simulink model "ControlSystemSimulation"  (R2023a)
settings: Solver=FixedStepDiscrete  StartTime=0.0  StopTime=60  FixedStep=Ts  RelTol=1e-3
undefined symbols (not defined in the file): A_eso, Aa, Ad, b0, B_eso, Ba, Bd, C_eso, Ca, Cd, D_eso, deltaAd, deltay, DiscIntNeverNeededParam, Ed, k_current, k_disturb, k_MN, k_of, Kc, L, N, nr, p_MN, p_of, T, Ts, vmax, wsin, z_MN, z_of
libraries: simulink x5, cstblocks x4, slpidlib x2
settings Model: Creator=jueqi  LastModifiedBy=13529

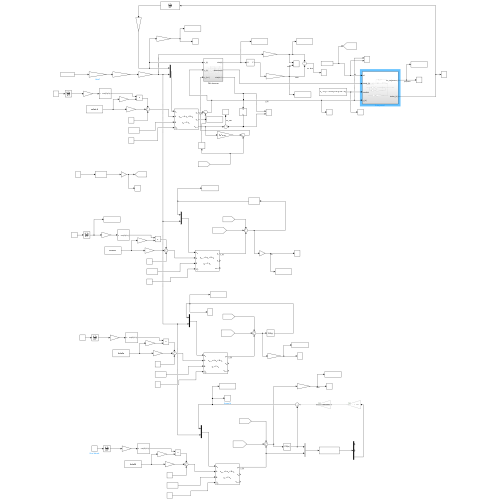
[thumbnail: Simulink's stored preview of the top-level diagram]
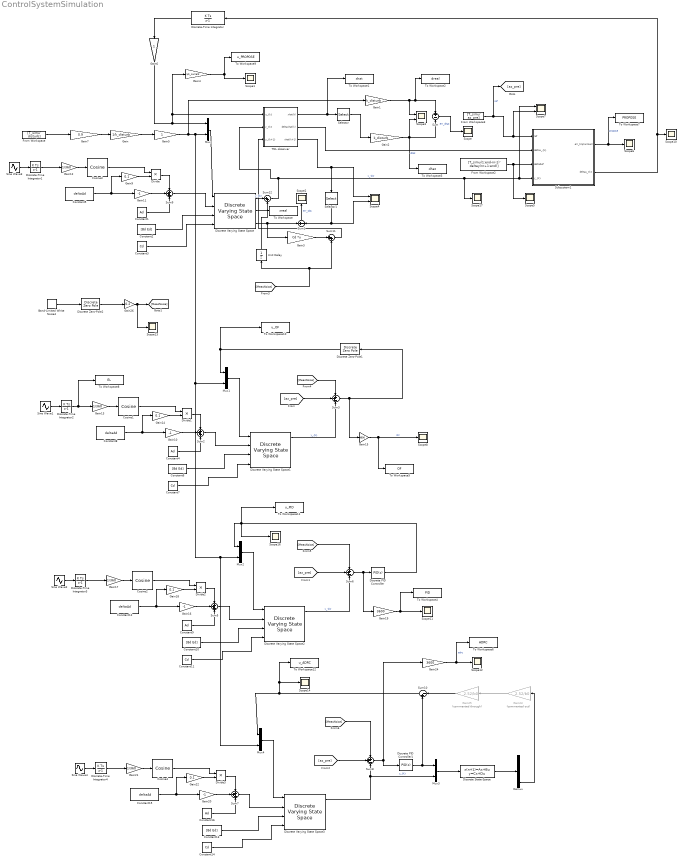
== system ControlSystemSimulation ==
  Band-Limited White Noise4 : simulink/Sources/Band-Limited White Noise  Cov=[1e-12]  Ts=Ts  seed=[23341]
  Constant{1,4,9,16} (4 alike) : Constant  Value=Ad
  Constant{2,6,10,13} (4 alike) : Constant  Value=[Bd Ed]
  Constant{3,7,11,14} (4 alike) : Constant  Value=Cd  VectorParams1D=off
  Constant{5,8,12,15} (4 alike) : Constant  Value=deltaAd
  Cosine{1..4} (4 alike) : simulink/Lookup Tables/Cosine  Formula=cos(2*pi*u)  NumDataPoints=(2^5)+1  OutputWordLength=16  InternalRulePriority=Speed
  Demux : Demux  Outputs=3
  Discrete Zero-Pole1 : DiscreteZeroPole  Zeros=z_of  Poles=p_of  Gain=k_of  SampleTime=Ts
  Discrete Zero-Pole2 : DiscreteZeroPole  Zeros=z_MN  Poles=p_MN  Gain=k_MN  SampleTime=Ts
  Discrete PID Controller : slpidlib/PID Controller  Controller=PID  Form=Parallel  TimeDomain=Discrete-time  UseExternalTs=off  SampleTime=-1  IntegratorMethod=Forward Euler  FilterMethod=Forward Euler  ControllerParametersSource=internal  P=25  I=0.3  UseKiTs=off  D=5  N=100  UseFilter=on  TunerSelectOption=Transfer Function Based (PID Tuner App)  InitialConditionSource=internal  InitialConditionForIntegrator=0  InitialConditionForFilter=0  DifferentiatorICPrevScaledInput=0  ExternalReset=none  TrackingMode=off  Kt=1  LimitOutput=off  SatLimitsSource=internal  UpperSaturationLimit=inf  LowerSaturationLimit=-inf  LinearizeAsGain=off  AntiWindupMode=none  Kb=1  LimitIntegrator=off  UpperIntegratorSaturationLimit=inf  LowerIntegratorSaturationLimit=-inf  POutMin=[]  POutMax=[]  IOutMin=[]  IOutMax=[]  DOutMin=[]  DOutMax=[]  NOutMin=[]  NOutMax=[]  SumOutMin=[]  SumOutMax=[]  SaturationOutMin=[]  SaturationOutMax=[]  PParamMin=[]  PParamMax=[]  IParamMin=[]  IParamMax=[]  DParamMin=[]  DParamMax=[]  NParamMin=[]  NParamMax=[]  KbParamMin=[]  KbParamMax=[]  KtParamMin=[]  KtParamMax=[]  KbOutMin=[]  KbOutMax=[]  KtOutMin=[]  KtOutMax=[]  IntegratorOutMin=[]  IntegratorOutMax=[]  FilterOutMin=[]  FilterOutMax=[]  SumI1OutMin=[]  SumI1OutMax=[]  SumI2OutMin=[]  SumI2OutMax=[]  SumI3OutMin=[]  SumI3OutMax=[]  SumI4OutMin=[]  SumI4OutMax=[]  SumDOutMin=[]  SumDOutMax=[]  DifferentiatorOutMin=[]  DifferentiatorOutMax=[]  FilterDiffOutCoefMin=[]  FilterDiffOutCoefMax=[]  ReciprocalOutMin=[]  ReciprocalOutMax=[]  SumDenOutMin=[]  SumDenOutMax=[]  SumNumOutMin=[]  SumNumOutMax=[]  DivideOutMin=[]  DivideOutMax=[]  UdiffTsProdOutMin=[]  UdiffTsProdOutMax=[]  NTsProdOutMin=[]  NTsProdOutMax=[]  UintegralTsProdOutMin=[]  UintegralTsProdOutMax=[]  UngainTsProdOutMin=[]  UngainTsProdOutMax=[]  ClampingZeroOutDataTypeStr=Inherit: Inherit via back propagation  ClampingZeroOutMin=[]  ClampingZeroOutMax=[]  FilterDenConstantOutDataTypeStr=Inherit: Inherit via back propagation  FilterDenConstantOutMin=[]  FilterDenConstantOutMax=[]  PCopyOutDataTypeStr=Inherit: Inherit via back propagation  PCopyOutMin=[]  PCopyOutMax=[]  NCopyOutDataTypeStr=Inherit: Inherit via back propagation  NCopyOutMin=[]  NCopyOutMax=[]  IntegratorContinuousStateAttributes=''  IntegratorStateMustResolveToSignalObject=off  IntegratorRTWStateStorageClass=Auto  FilterContinuousStateAttributes=''  FilterStateMustResolveToSignalObject=off  FilterRTWStateStorageClass=Auto  ParallelPVariant=InternalParameters  IdealPVariant=Disabled  IVariant=InternalParameters  DVariant=InternalParameters  IntegratorVariant=Discrete  SatVariant=Disabled  AWVariant=Passthrough  PCopyVariant=Disabled  TRVariant=Disabled  FdbkBlocksVariant=Forward  IdealPFdbkVariant=Disabled  SatFdbkVariant=Disabled  DerivativeFilterVariant=ForwardEulerFilter  NVariant=InternalParameters  NCopyVariant=Disabled  FilterICVariant=InternalICsFilter  IntegratorICVariant=InternalICs  ExternalResetVariant=Disabled  TRSumVariant=Passthrough  SumFdbkVariant=Disabled  SumVariant=Sum_PID  TsampFilterVariant=InternalTs  TsampNgainVariant=Passthrough  TsampIntegralVariant=Disabled_SignalSpec  ExternalSaturationOutDataTypeStr=Inherit: Same as second input
      settings: LibrarySourceBlock=simulink/Discrete/Discrete PID Controller
  Discrete PID Controller1 : slpidlib/PID Controller  Controller=PID  Form=Parallel  TimeDomain=Discrete-time  UseExternalTs=off  SampleTime=-1  IntegratorMethod=Forward Euler  FilterMethod=Forward Euler  ControllerParametersSource=internal  P=150  I=1  UseKiTs=off  D=15  N=100  UseFilter=on  TunerSelectOption=Transfer Function Based (PID Tuner App)  InitialConditionSource=internal  InitialConditionForIntegrator=0  InitialConditionForFilter=0  DifferentiatorICPrevScaledInput=0  ExternalReset=none  TrackingMode=off  Kt=1  LimitOutput=off  SatLimitsSource=internal  UpperSaturationLimit=inf  LowerSaturationLimit=-inf  LinearizeAsGain=off  AntiWindupMode=none  Kb=1  LimitIntegrator=off  UpperIntegratorSaturationLimit=inf  LowerIntegratorSaturationLimit=-inf  POutMin=[]  POutMax=[]  IOutMin=[]  IOutMax=[]  DOutMin=[]  DOutMax=[]  NOutMin=[]  NOutMax=[]  SumOutMin=[]  SumOutMax=[]  SaturationOutMin=[]  SaturationOutMax=[]  PParamMin=[]  PParamMax=[]  IParamMin=[]  IParamMax=[]  DParamMin=[]  DParamMax=[]  NParamMin=[]  NParamMax=[]  KbParamMin=[]  KbParamMax=[]  KtParamMin=[]  KtParamMax=[]  KbOutMin=[]  KbOutMax=[]  KtOutMin=[]  KtOutMax=[]  IntegratorOutMin=[]  IntegratorOutMax=[]  FilterOutMin=[]  FilterOutMax=[]  SumI1OutMin=[]  SumI1OutMax=[]  SumI2OutMin=[]  SumI2OutMax=[]  SumI3OutMin=[]  SumI3OutMax=[]  SumI4OutMin=[]  SumI4OutMax=[]  SumDOutMin=[]  SumDOutMax=[]  DifferentiatorOutMin=[]  DifferentiatorOutMax=[]  FilterDiffOutCoefMin=[]  FilterDiffOutCoefMax=[]  ReciprocalOutMin=[]  ReciprocalOutMax=[]  SumDenOutMin=[]  SumDenOutMax=[]  SumNumOutMin=[]  SumNumOutMax=[]  DivideOutMin=[]  DivideOutMax=[]  UdiffTsProdOutMin=[]  UdiffTsProdOutMax=[]  NTsProdOutMin=[]  NTsProdOutMax=[]  UintegralTsProdOutMin=[]  UintegralTsProdOutMax=[]  UngainTsProdOutMin=[]  UngainTsProdOutMax=[]  ClampingZeroOutDataTypeStr=Inherit: Inherit via back propagation  ClampingZeroOutMin=[]  ClampingZeroOutMax=[]  FilterDenConstantOutDataTypeStr=Inherit: Inherit via back propagation  FilterDenConstantOutMin=[]  FilterDenConstantOutMax=[]  PCopyOutDataTypeStr=Inherit: Inherit via back propagation  PCopyOutMin=[]  PCopyOutMax=[]  NCopyOutDataTypeStr=Inherit: Inherit via back propagation  NCopyOutMin=[]  NCopyOutMax=[]  IntegratorContinuousStateAttributes=''  IntegratorStateMustResolveToSignalObject=off  IntegratorRTWStateStorageClass=Auto  FilterContinuousStateAttributes=''  FilterStateMustResolveToSignalObject=off  FilterRTWStateStorageClass=Auto  ParallelPVariant=InternalParameters  IdealPVariant=Disabled  IVariant=InternalParameters  DVariant=InternalParameters  IntegratorVariant=Discrete  SatVariant=Disabled  AWVariant=Passthrough  PCopyVariant=Disabled  TRVariant=Disabled  FdbkBlocksVariant=Forward  IdealPFdbkVariant=Disabled  SatFdbkVariant=Disabled  DerivativeFilterVariant=ForwardEulerFilter  NVariant=InternalParameters  NCopyVariant=Disabled  FilterICVariant=InternalICsFilter  IntegratorICVariant=InternalICs  ExternalResetVariant=Disabled  TRSumVariant=Passthrough  SumFdbkVariant=Disabled  SumVariant=Sum_PID  TsampFilterVariant=InternalTs  TsampNgainVariant=Passthrough  TsampIntegralVariant=Disabled_SignalSpec  ExternalSaturationOutDataTypeStr=Inherit: Same as second input
      settings: LibrarySourceBlock=simulink/Discrete/Discrete PID Controller
  Discrete State-Space : DiscreteStateSpace  A=A_eso  B=B_eso  C=C_eso  D=D_eso  SampleTime=Ts
  Discrete Varying State Space{,1..3} (4 alike) : cstblocks/Linear Parameter Varying/Discrete Varying State Space  x0=[0 0 0 0 0]  Ts=Ts  OutputX=on  OutputDX=on  Feedthrough=off
  Discrete-Time Integrator : DiscreteIntegrator  gainval=Fs  SampleTime=Ts  UpperSaturationLimit=500  LowerSaturationLimit=-500  ICPrevOutput=DiscIntNeverNeededParam  ICPrevScaledInput=DiscIntNeverNeededParam
  Discrete-Time Integrator{1..4} (4 alike) : DiscreteIntegrator  SampleTime=-1  ICPrevOutput=DiscIntNeverNeededParam  ICPrevScaledInput=DiscIntNeverNeededParam
  Divide{,1..3} (4 alike) : Product  Inputs=**
  From Workspace : FromWorkspace  VariableName=[T_simu' disturb]  SampleTime=Ts
  From Workspace2 : FromWorkspace  VariableName=[T_simu(1:end-nr-1)' deltay(nr+1:end)]  SampleTime=Ts
  From Workspace3 : FromWorkspace  VariableName=[T_simu' az_pre]
  Gain : Gain  Gain=1/k_disturb
  Gain1 : Gain  Gain=k_disturb
  Gain{10..11,16,20} (4 alike) : Gain  Gain=-1
  Gain{12..13,17,21} (4 alike) : Gain  Gain=1/360
  Gain{9,14,18,22} (4 alike) : Gain  Gain=0.1
  Gain15 : Gain  Gain=3600
  Gain19 : Gain  Gain=3600
  Gain2 : Gain  Gain=k_disturb
  Gain23 : Gain  Commented=on  Gain=2.52/b0
  Gain24 : Gain  Gain=3600
  Gain25 : Gain  Commented=through  Gain=2.52/b0
  Gain26 : Gain  Gain=0.2
  Gain3 : Gain  Gain=Cd  Multiplication=Matrix(K*u) (u vector)
  Gain4 : Gain  Gain=1/k_current
  Gain5 : Gain
  Gain6 : Gain
  Gain7 : Gain  Gain=0.9
  Mux{,1..4} (5 alike) : Mux  Inputs=2
  Scope{,1..2,5..6,8,10..14,16..17} (13 alike) : Scope
  Scope3 : Scope  NumInputPorts=2
  Scope4 : Scope  NumInputPorts=2
  Scope7 : Scope  NumInputPorts=2
  Selector : Selector  InputPortWidth=6  IndexOptions=Index vector (dialog)  Indices=[6]  OutputSizes=1
  Selector1 : Selector  InputPortWidth=6  IndexOptions=Index vector (dialog)  Indices=[1:5]  OutputSizes=1
  Sine Wave{1..4} (4 alike) : Sin  Amplitude=vmax  Bias=vmax  Frequency=wsin  Phase=3/2*pi  SampleTime=Ts
  Subsystem1 : Subsystem
  Sum : Sum  Inputs=+|-
  Sum1 : Sum  Inputs=+|-
  Sum10 : Sum  Inputs=|-+
  Sum11 : Sum  Inputs=|++
  Sum12 : Sum  Inputs=|++
  Sum{2,5,7,9} (4 alike) : Sum  Inputs=+++
  Sum3 : Sum  Inputs=++-
  Sum6 : Sum  Inputs=++-
  Sum8 : Sum  Inputs=++-
  TNL observer : Subsystem
  To Workspace : ToWorkspace  VariableName=xreal  SampleTime=Ts
  To Workspace1 : ToWorkspace  VariableName=xhat  SampleTime=Ts
  To Workspace10 : ToWorkspace  VariableName=u_OF  SampleTime=Ts
  To Workspace11 : ToWorkspace  VariableName=u_PID  SampleTime=Ts
  To Workspace12 : ToWorkspace  VariableName=u_ADRC  SampleTime=Ts
  To Workspace2 : ToWorkspace  VariableName=dreal  SampleTime=Ts
  To Workspace3 : ToWorkspace  VariableName=dhat  SampleTime=Ts
  To Workspace4 : ToWorkspace  VariableName=PID  SampleTime=Ts
  To Workspace5 : ToWorkspace  VariableName=OF  SampleTime=Ts
  To Workspace6 : ToWorkspace  VariableName=ADRC  SampleTime=Ts
  To Workspace7 : ToWorkspace  VariableName=PROPOSE  SampleTime=Ts
  To Workspace8 : ToWorkspace  VariableName=EL  SampleTime=Ts
  To Workspace9 : ToWorkspace  VariableName=u_PROPOSE  SampleTime=Ts
  Unit Delay : UnitDelay  SampleTime=Ts  HasFrameUpgradeWarning=on
  wires:
  Gain9/1 -> Divide/2
  Gain11/1 -> Sum9/2
  Divide/1 -> Sum9/1
  Constant1/1 -> Sum9/3
  Mux/1 -> Discrete Varying State Space/1
  TNL observer/2(deltaxhat(k)) -> Subsystem1/2("deltax_{k}")
  Subsystem1/2("deltau_{k}") -> Scope10/1, Discrete-Time Integrator/1
  Sum11/1 -> TNL observer/3("y_{k+1}")
  Selector/1 -> Gain2/1
  Sum12/1 -> TNL observer/2("y_{k}"), Scope17/1, Scope7/1, Subsystem1/4("y_{k}")  "y_{k}"
  Sum1/1 -> Scope2/1  "err_obs"
  From Workspace3/1 -> [az_pre], Scope7/2, Subsystem1/1(ref)  "ref"
  Discrete-Time Integrator/1 -> Gain6/1
  Discrete Varying State Space/3 -> Gain3/1, Sum1/1
  Subsystem1/1(err_traj(arcsec)) -> To Workspace7/1, Scope6/1  "propose"
  Gain7/1 -> Gain/1
  Sum9/1 -> Discrete Varying State Space/2
  Constant2/1 -> Discrete Varying State Space/3
  TNL observer/3(xhat(k+1)) -> Scope4/1, Selector1/1
  From Workspace/1 -> Gain7/1
  Selector1/1 -> Scope4/2, Sum1/2
  From Workspace2/1 -> Scope5/1, Subsystem1/3(deltaRef)
  Sum/1 -> Scope/1  "err_dhat"
  Gain2/1 -> Scope3/2, To Workspace3/1, Sum/2  "dhat"
  Gain/1 -> Gain5/1
  Constant5/1 -> Gain11/1, Gain9/1
  Constant3/1 -> Discrete Varying State Space/4
  Sine Wave3/1 -> Discrete-Time Integrator1/1
  Gain12/1 -> Cosine3/1
  Discrete-Time Integrator1/1 -> Gain12/1
  Cosine3/1 -> Divide/1
  Gain1/1 -> To Workspace2/1, Sum/1, Scope3/1
  TNL observer/1(xhat(k)) -> To Workspace1/1, Selector/1
  Discrete Varying State Space/2 -> To Workspace/1
  Cosine1/1 -> Divide1/1
  Discrete-Time Integrator2/1 -> To Workspace8/1, Gain13/1
  Gain13/1 -> Cosine1/1
  Sine Wave1/1 -> Discrete-Time Integrator2/1
  Constant7/1 -> Discrete Varying State Space1/4
  Constant8/1 -> Gain14/1, Gain10/1
  Constant6/1 -> Discrete Varying State Space1/3
  Sum2/1 -> Discrete Varying State Space1/2
  Mux1/1 -> Discrete Varying State Space1/1
  Constant4/1 -> Sum2/3
  Divide1/1 -> Sum2/1
  Gain10/1 -> Sum2/2
  Gain14/1 -> Divide1/2
  Discrete Varying State Space1/1 -> Sum3/3  "y_{k}"
  [az_pre] -> Sum3/2
  Sum3/1 -> Discrete Zero-Pole1/1, Gain15/1
  Gain15/1 -> To Workspace5/1, Scope8/1  "OF"
  Gain19/1 -> To Workspace4/1, Scope11/1
  Sum6/1 -> Discrete PID Controller/1, Gain19/1
  [az_pre] -> Sum6/2
  Discrete Varying State Space2/1 -> Sum6/3  "y_{k}"
  Gain18/1 -> Divide2/2
  Gain16/1 -> Sum5/2
  Divide2/1 -> Sum5/1
  Constant9/1 -> Sum5/3
  Mux2/1 -> Discrete Varying State Space2/1
  Sum5/1 -> Discrete Varying State Space2/2
  Constant10/1 -> Discrete Varying State Space2/3
  Constant12/1 -> Gain16/1, Gain18/1
  Constant11/1 -> Discrete Varying State Space2/4
  Sine Wave2/1 -> Discrete-Time Integrator3/1
  Gain17/1 -> Cosine2/1
  Discrete-Time Integrator3/1 -> Gain17/1
  Cosine2/1 -> Divide2/1
  [MeasNoise] -> Sum6/1
  [MeasNoise] -> Sum3/1
  Discrete Zero-Pole1/1 -> To Workspace10/1, Mux1/1
  Mux3/1 -> Discrete State-Space/1
  [MeasNoise] -> Sum8/1
  Gain5/1 -> Gain1/1, Mux1/2, Mux4/2, Mux2/2, Mux/2
  Cosine4/1 -> Divide3/1
  Discrete-Time Integrator4/1 -> Gain21/1
  Gain21/1 -> Cosine4/1
  Sine Wave4/1 -> Discrete-Time Integrator4/1
  Constant14/1 -> Discrete Varying State Space3/4
  Constant15/1 -> Gain22/1, Gain20/1
  Constant13/1 -> Discrete Varying State Space3/3
  Sum7/1 -> Discrete Varying State Space3/2
  Mux4/1 -> Discrete Varying State Space3/1
  Constant16/1 -> Sum7/3
  Divide3/1 -> Sum7/1
  Gain20/1 -> Sum7/2
  Gain22/1 -> Divide3/2
  Discrete Varying State Space3/1 -> Mux3/2, Sum8/3  "y_{k}"
  [az_pre] -> Sum8/2
  Sum8/1 -> Discrete PID Controller1/1, Gain24/1
  Discrete State-Space/1 -> Demux/1
  Sum10/1 -> Scope14/1, To Workspace12/1, Mux4/1
  Discrete PID Controller1/1 -> Mux3/1, Sum10/2
  Gain23/1 -> Gain25/1
  Demux/3 -> Gain23/1
  Gain24/1 -> To Workspace6/1, Scope12/1  "adrc"
  Gain25/1 -> Sum10/1
  Discrete PID Controller/1 -> Scope16/1, To Workspace11/1, Mux2/1
  Gain3/1 -> Sum11/1
  [MeasNoise] -> Unit Delay/1, Sum11/2
  Discrete Varying State Space/1 -> Sum12/1  "y_{k}"
  Unit Delay/1 -> Sum12/2
  Band-Limited White Noise4/1 -> Discrete Zero-Pole2/1
  Discrete Zero-Pole2/1 -> Gain26/1
  Gain26/1 -> Scope13/1, [MeasNoise]
  Gain4/1 -> Scope1/1, To Workspace9/1
  Gain6/1 -> TNL observer/1("u_{k}"), Gain4/1, Mux/1

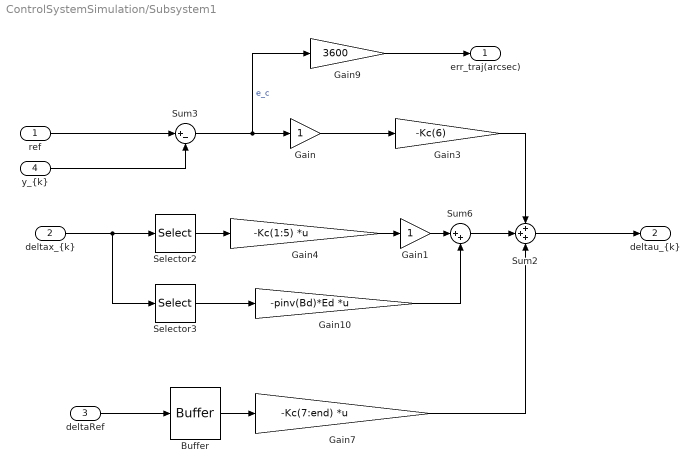
== system ControlSystemSimulation/Subsystem1 ==
  ref : Inport
  "deltax_{k}" : Inport  Port=2
  deltaRef : Inport  Port=3
  "y_{k}" : Inport  Port=4
  Buffer : Buffer  N=nr  V=nr-1  ic=deltay(1:nr)  OutputFrames=off
  Gain : Gain
  Gain1 : Gain
  Gain10 : Gain  Gain=-pinv(Bd)*Ed  Multiplication=Matrix(K*u) (u vector)
  Gain3 : Gain  Gain=-Kc(6)
  Gain4 : Gain  Gain=-Kc(1:5)  Multiplication=Matrix(K*u) (u vector)
  Gain7 : Gain  Gain=-Kc(7:end)  Multiplication=Matrix(K*u) (u vector)
  Gain9 : Gain  Gain=3600
  Selector2 : Selector  InputPortWidth=6  IndexOptions=Index vector (dialog)  Indices=[1:5]  OutputSizes=1
  Selector3 : Selector  InputPortWidth=6  IndexOptions=Index vector (dialog)  Indices=[6]  OutputSizes=1
  Sum2 : Sum  Inputs=+++
  Sum3 : Sum  Inputs=|+-
  Sum6 : Sum  Inputs=|++
  err_traj(arcsec) : Outport
  "deltau_{k}" : Outport  Port=2
  wires:
  Selector2/1 -> Gain4/1
  Gain3/1 -> Sum2/1
  Sum3/1 -> Gain/1, Gain9/1  "e_c"
  Selector3/1 -> Gain10/1
  Gain4/1 -> Gain1/1
  Gain10/1 -> Sum6/2
  Gain7/1 -> Sum2/3
  Sum6/1 -> Sum2/2
  "deltax_{k}"/1 -> Selector2/1, Selector3/1
  Buffer/1 -> Gain7/1
  Gain9/1 -> err_traj(arcsec)/1
  ref/1 -> Sum3/1
  "y_{k}"/1 -> Sum3/2
  deltaRef/1 -> Buffer/1
  Gain/1 -> Gain3/1
  Sum2/1 -> "deltau_{k}"/1
  Gain1/1 -> Sum6/1

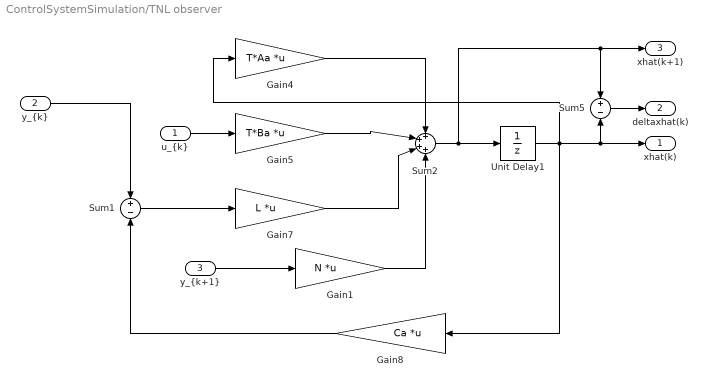
== system ControlSystemSimulation/TNL observer ==
  "u_{k}" : Inport
  "y_{k}" : Inport  Port=2
  "y_{k+1}" : Inport  Port=3
  Gain1 : Gain  Gain=N  Multiplication=Matrix(K*u) (u vector)
  Gain4 : Gain  Gain=T*Aa  Multiplication=Matrix(K*u) (u vector)
  Gain5 : Gain  Gain=T*Ba  Multiplication=Matrix(K*u) (u vector)
  Gain7 : Gain  Gain=L  Multiplication=Matrix(K*u) (u vector)
  Gain8 : Gain  Gain=Ca  Multiplication=Matrix(K*u) (u vector)
  Sum1 : Sum  Inputs=+|-
  Sum2 : Sum  Inputs=++++
  Sum5 : Sum  Inputs=+|-
  Unit Delay1 : UnitDelay  InitialCondition=[0 0 0 0 0 0]  SampleTime=Ts  HasFrameUpgradeWarning=on
  xhat(k) : Outport
  deltaxhat(k) : Outport  Port=2
  xhat(k+1) : Outport  Port=3
  wires:
  Sum2/1 -> Sum5/1, xhat(k+1)/1, Unit Delay1/1
  Gain4/1 -> Sum2/1
  Sum1/1 -> Gain7/1
  Gain5/1 -> Sum2/2
  Gain7/1 -> Sum2/3
  Gain8/1 -> Sum1/2
  "y_{k}"/1 -> Sum1/1
  "u_{k}"/1 -> Gain5/1
  Unit Delay1/1 -> Gain8/1, xhat(k)/1, Sum5/2, Gain4/1
  Sum5/1 -> deltaxhat(k)/1
  "y_{k+1}"/1 -> Gain1/1
  Gain1/1 -> Sum2/4
